simulink model "pi_control"  (R2026a)
settings: Solver=FixedStepAuto  StopTime=inf  EnableMultiTasking=on
undefined symbols (not defined in the file): dspblkCoreblockFVToolHelper, gcbh
libraries: arduinosensorlib x1, slpidlib x1, arduinolib x1
settings Model: SILPILModeSetting=veronly  ExtModeTrigDuration=2  Creator=cas_g  LastModifiedBy=00782620
settings HardwareCC: ProdBitPerInt=16.0  ProdBitPerPointer=16.0  ProdBitPerSizeT=16.0  ProdBitPerPtrDiffT=16.0  ProdWordSize=8.0  ProdHWDeviceType=Atmel->AVR
settings RTWCC: SystemTargetFile=ert.tlc  HardwareBoard=Arduino Uno  TLCOptions=-aInlineSetEventsForThisBaseRateFcn=TLC_FALSE -aSuppressMultiTaskScheduler=TLC_FALSE -aRateBasedStepFcn=1  Toolchain=Arduino AVR  BuildConfiguration=Faster Runs  Description=Embedded Coder
settings ERTTargetCC: ExtModeTransport=3.0  ExtModeAutomaticAllocSize=off  ExtModeStaticAllocSize=250.0  SupportContinuousTime=on  SupportVariableSizeSignals=on

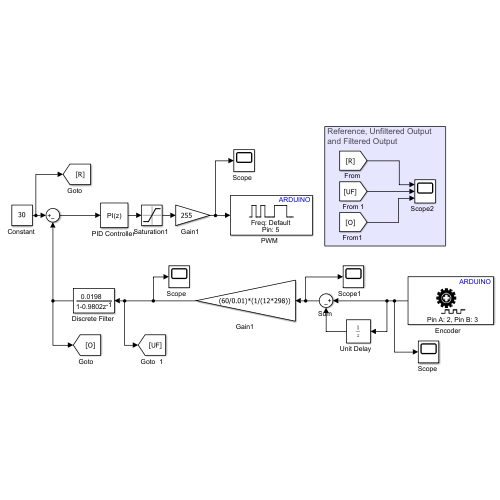
[thumbnail: Simulink's stored preview of the top-level diagram]
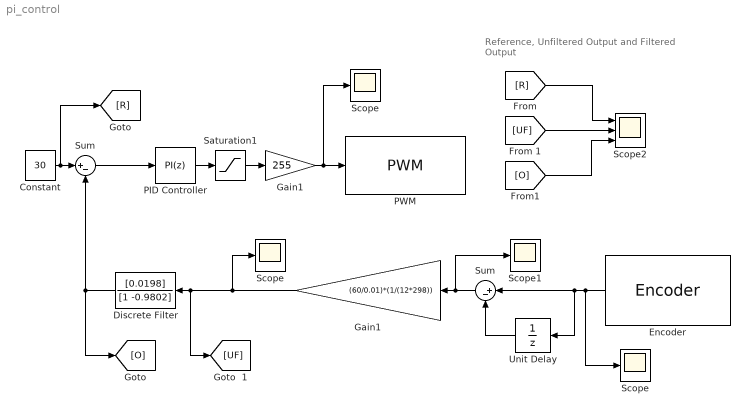
== system pi_control ==
  note: Reference, Unfiltered Output
      | and Filtered Output
  "Constant " : Constant  Value=30
  "Discrete Filter " : DiscreteFilter  LoadFcn=dspblkCoreblockFVToolHelper(gcbh,'load');  Numerator=[0.0198]  Denominator=[1 -0.9802]
      settings: CopyFcn=dspblkCoreblockFVToolHelper(gcbh,'copy');  DeleteFcn=dspblkCoreblockFVToolHelper(gcbh,'close');  ModelCloseFcn=dspblkCoreblockFVToolHelper(gcbh,'close');  PreSaveFcn=dspblkCoreblockFVToolHelper(gcbh,'presave');  PostSaveFcn=dspblkCoreblockFVToolHelper(gcbh,'postsave');  CloseFcn=dspblkCoreblockFVToolHelper(gcbh,'close');
  "Encoder   " : arduinosensorlib/Encoder  InputA=2  InputB=3  Mode=No reset  SampleTime=0.01
  "Gain1 " : Gain  Gain=(60/0.01)*(1/(12*298))
  "Gain1   " : Gain  Gain=255
  "PID Controller " : slpidlib/PID Controller  Controller=PI  Form=Parallel  TimeDomain=Discrete-time  UseExternalTs=off  SampleTime=0.01  IntegratorMethod=Backward Euler  FilterMethod=Forward Euler  ControllerParametersSource=internal  P=0.1  I=0.05  UseKiTs=off  D=0  UseExternalDerivativeSource=off  N=100  UseFilter=on  TunerSelectOption=Transfer Function Based (PID Tuner App)  InitialConditionSource=internal  InitialConditionForIntegrator=0  InitialConditionForFilter=0  DifferentiatorICPrevScaledInput=0  ExternalReset=none  TrackingMode=off  Kt=1  LimitOutput=off  SatLimitsSource=internal  UpperSaturationLimit=inf  LowerSaturationLimit=-inf  LinearizeAsGain=on  AntiWindupMode=none  Kb=1  LimitIntegrator=off  UpperIntegratorSaturationLimit=inf  LowerIntegratorSaturationLimit=-inf  POutMin=[]  POutMax=[]  IOutMin=[]  IOutMax=[]  DOutMin=[]  DOutMax=[]  NOutMin=[]  NOutMax=[]  SumOutMin=[]  SumOutMax=[]  SaturationOutMin=[]  SaturationOutMax=[]  PParamMin=[]  PParamMax=[]  IParamMin=[]  IParamMax=[]  DParamMin=[]  DParamMax=[]  NParamMin=[]  NParamMax=[]  KbParamMin=[]  KbParamMax=[]  KtParamMin=[]  KtParamMax=[]  KbOutMin=[]  KbOutMax=[]  KtOutMin=[]  KtOutMax=[]  IntegratorOutMin=[]  IntegratorOutMax=[]  FilterOutMin=[]  FilterOutMax=[]  SumI1OutMin=[]  SumI1OutMax=[]  SumI2OutMin=[]  SumI2OutMax=[]  SumI3OutMin=[]  SumI3OutMax=[]  SumI4OutMin=[]  SumI4OutMax=[]  SumDOutMin=[]  SumDOutMax=[]  DifferentiatorOutMin=[]  DifferentiatorOutMax=[]  FilterDiffOutCoefMin=[]  FilterDiffOutCoefMax=[]  ReciprocalOutMin=[]  ReciprocalOutMax=[]  SumDenOutMin=[]  SumDenOutMax=[]  SumNumOutMin=[]  SumNumOutMax=[]  DivideOutMin=[]  DivideOutMax=[]  UdiffTsProdOutMin=[]  UdiffTsProdOutMax=[]  NTsProdOutMin=[]  NTsProdOutMax=[]  UintegralTsProdOutMin=[]  UintegralTsProdOutMax=[]  UngainTsProdOutMin=[]  UngainTsProdOutMax=[]  ClampingZeroOutDataTypeStr=Inherit: Inherit via back propagation  ClampingZeroOutMin=[]  ClampingZeroOutMax=[]  FilterDenConstantOutDataTypeStr=Inherit: Inherit via back propagation  FilterDenConstantOutMin=[]  FilterDenConstantOutMax=[]  PCopyOutDataTypeStr=Inherit: Inherit via back propagation  PCopyOutMin=[]  PCopyOutMax=[]  NCopyOutDataTypeStr=Inherit: Inherit via back propagation  NCopyOutMin=[]  NCopyOutMax=[]  IntegratorContinuousStateAttributes=''  IntegratorStateMustResolveToSignalObject=off  IntegratorRTWStateStorageClass=Auto  FilterContinuousStateAttributes=''  FilterStateMustResolveToSignalObject=off  FilterRTWStateStorageClass=Auto  ParallelPVariant=InternalParameters  IdealPVariant=Disabled  IVariant=InternalParameters  DVariant=Disabled  IntegratorVariant=Discrete  SatVariant=Disabled  AWVariant=Passthrough  PCopyVariant=Disabled  TRVariant=Disabled  FdbkBlocksVariant=Forward  IdealPFdbkVariant=Disabled  SatFdbkVariant=Disabled  DerivativeFilterVariant=Disabled  NVariant=Disabled  NCopyVariant=Disabled_SignalSpec  FilterICVariant=Disabled  IntegratorICVariant=InternalICs  ExternalResetVariant=Disabled  TRSumVariant=Passthrough  SumFdbkVariant=Disabled  SumVariant=Sum_PI  TsampFilterVariant=InternalTs  TsampNgainVariant=Passthrough  TsampIntegralVariant=Disabled_SignalSpec  ExternalSaturationOutDataTypeStr=Inherit: Same as second input  DerivativeSourceVariant=Disabled  PreIntVariant=InternalPreInt
  "PWM  " : arduinolib/PWM  pinNumber=5  frequencyType=Default  desiredFrequency=490.2  achievableFrequency=490.2
  "Saturation1 " : Saturate  UpperLimit=1  LowerLimit=-1
  "Scope " : Scope
      settings: ActiveDisplayYMinimum=-2.3831591275E+9  ActiveDisplayYMaximum=1.3459963075E+9
  "Scope  " : Scope
      settings: ActiveDisplayYMinimum=-318.75  ActiveDisplayYMaximum=318.75
  "Scope   " : Scope
      settings: ActiveDisplayYMinimum=-8.1795302031096053  ActiveDisplayYMaximum=56.837248334428295  DataLoggingVariableName=ScopeData4
  "Scope1    " : Scope
      settings: ActiveDisplayYMinimum=-2.2499999999999996  ActiveDisplayYMaximum=20.25  DataLoggingVariableName=ScopeData5
  "Scope2   " : Scope  NumInputPorts=3
      settings: ActiveDisplayYMinimum=-3.7499999999999991  ActiveDisplayYMaximum=33.75  DataLoggingVariableName=ScopeData2
  Sum : Sum  Inputs=|+-
  "Sum " : Sum  Inputs=|+-
  "Unit Delay   " : UnitDelay  SampleTime=-1
  wires:
  [R] -> "Scope2   "/1
  [O] -> "Scope2   "/3
  "Sum "/1 -> "Scope1    "/1, "Gain1 "/1
  "Unit Delay   "/1 -> "Sum "/2
  "Discrete Filter "/1 -> Sum/2, [O]
  "Constant "/1 -> [R], Sum/1
  Sum/1 -> "PID Controller "/1
  "PID Controller "/1 -> "Saturation1 "/1
  "Saturation1 "/1 -> "Gain1   "/1
  "Gain1   "/1 -> "Scope  "/1, "PWM  "/1
  [UF] -> "Scope2   "/2
  "Encoder   "/1 -> "Scope "/1, "Sum "/1, "Unit Delay   "/1
  "Gain1 "/1 -> "Discrete Filter "/1, [UF], "Scope   "/1
